simulink model "CombinedExperiment"  (R2020a)
settings: Solver=FixedStepAuto  StartTime=0.0  StopTime=tsim  FixedStep=baseRate  RelTol=1e-3  EnableMultiTasking=on
values from neighbouring files (symbols this model uses):
  baseRate = 0.1    [Run_Initializer.m]
  drop_states_BLACK = [1.36947387695313,1.22175756835938,-0.0161599479615688]    [Run_Initializer.m]
  drop_states_BLUE = [ xLength/2+0.9; yLength/2+0.5; 0]    [Run_Initializer.m]
  drop_states_RED = [ xLength/2+1.1; yLength/2; pi]    [Run_Initializer.m]
  F_thrusters_BLACK = 0.25.*ones(8,1)    [Run_Initializer.m]
  F_thrusters_BLUE = 0.25.*ones(8,1)    [Run_Initializer.m]
  F_thrusters_RED = 0.25.*ones(8,1)    [Run_Initializer.m]
  home_states_BLACK = [ xLength/2; yLength/2; 0]    [Run_Initializer.m]
  home_states_BLUE = [ xLength/2-0.9; yLength/2+0.5; 0]    [Run_Initializer.m]
  home_states_RED = [ xLength/2+1.1; yLength/2; pi]    [Run_Initializer.m]
  init_states_BLACK = [ xLength/2; yLength/2; 0]    [Run_Initializer.m]
  init_states_BLUE = [ xLength/2+0.9; yLength/2+0.5; 0]    [Run_Initializer.m]
  init_states_RED = [ xLength/2+1.1; yLength/2; pi]    [Run_Initializer.m]
  Kd_tb = 0.4    [Run_Initializer.m]
  Kd_tblue = 0.4    [Run_Initializer.m]
  Kd_tr = 0.4    [Run_Initializer.m]
  Kd_xb = 5    [Run_Initializer.m]
  Kd_xblue = 5    [Run_Initializer.m]
  Kd_xr = 5    [Run_Initializer.m]
  Kd_yb = 5    [Run_Initializer.m]
  Kd_yblue = 5    [Run_Initializer.m]
  Kd_yr = 5    [Run_Initializer.m]
  Kp_tb = 0.1    [Run_Initializer.m]
  Kp_tblue = 0.1    [Run_Initializer.m]
  Kp_tr = 0.1    [Run_Initializer.m]
  Kp_xb = 2    [Run_Initializer.m]
  Kp_xblue = 2    [Run_Initializer.m]
  Kp_xr = 2    [Run_Initializer.m]
  Kp_yb = 2    [Run_Initializer.m]
  Kp_yblue = 2    [Run_Initializer.m]
  Kp_yr = 2    [Run_Initializer.m]
  noise_variance_BLACK = 0    [Run_Initializer.m]
  noise_variance_BLUE = 0    [Run_Initializer.m]
  noise_variance_RED = 0    [Run_Initializer.m]
  Phase0_End = Phase0_Duration    (= 10)    [Run_Initializer.m]
  Phase1_End = Phase0_Duration + Phase1_Duration    (= 15)    [Run_Initializer.m]
  Phase2_End = Phase0_Duration + Phase1_Duration +                                   Phase2_Duration    (= 40)    [Run_Initializer.m]
  Phase3_End = Phase0_Duration + Phase1_Duration +                                   Phase2_Duration + Phase3_Duration    (= 117)    [Run_Initializer.m]
  Phase3_SubPhase1_End = Phase2_End + Phase3_SubPhase1_Duration    (= 41)    [Run_Initializer.m]
  Phase3_SubPhase2_End = Phase2_End + Phase3_SubPhase1_Duration +                                   Phase3_SubPhase2_Duration    (= 42)    [Run_Initializer.m]
  Phase3_SubPhase3_End = Phase2_End + Phase3_SubPhase1_Duration +                                   Phase3_SubPhase2_Duration +                                  Phase3_SubPhase3_Duration    (= 72)    [Run_Initializer.m]
  Phase3_SubPhase4_End = Phase2_End + Phase3_SubPhase1_Duration +                                   Phase3_SubPhase2_Duration +                                  Phase3_SubPhase3_Duration +                                  Phase3_SubPhase4_Duration    [Run_Initializer.m]
  Phase4_End = Phase0_Duration + Phase1_Duration +                                   Phase2_Duration + Phase3_Duration +                                   Phase4_Duration    (= 137)    [Run_Initializer.m]
  Phase5_End = Phase0_Duration + Phase1_Duration +                                   Phase2_Duration + Phase3_Duration +                                   Phase4_Duration + Phase5_Duration    (= 142)    [Run_Initializer.m]
  serverRate = 0.2    [Run_Initializer.m]
  thruster_dist2CG_BLACK = [83.42;-52.58;55.94;-60.05;54.08;-53.92;77.06;-55.94]    [Run_Initializer.m]
  thruster_dist2CG_BLUE = [83.42;-52.58;55.94;-60.05;54.08;-53.92;77.06;-55.94]    [Run_Initializer.m]
  thruster_dist2CG_RED = [49.92;-78.08;70.46;-63.54;81.08;-50.42;57.44;-75.96]    [Run_Initializer.m]
  xLength = 3.51155    [Run_Initializer.m]
  yLength = 2.41935    [Run_Initializer.m]
undefined symbols (not defined in the file or in its folder): DiscIntNeverNeededParam, platformSelection, simMode, WhoAmI
libraries: dspstat3 x18, raspberrypiBasiclib x10, dspsigops x9, embdlinuxlib x8, simulink x8, MainLibrary x5, mspfiltlib x3, dsparch4 x3, dspswit3 x2, sensehatlib x1
(part 4 of 9)

== system CombinedExperiment/From Force//Torque to PWM Signal/Change BLUE Behavior/Calculate Thruster ON//OFF ==
  note: Calculate which thrusters must be turned on and for how long.
  note: The H matrix is not square, thus a pserudo-inverse is required.
  note: Knowing how much force each thruster can output, we can determine the saturated thruster output and then convert is into a percentage of time over which each thruster is open.
  note: After finding the PWM value, we can use the H matrix to go back to torque and force. However, these torques and forces will be "saturated".
  "[Fx_b; Fy_b; Tz]" : Inport
  BLUE_Fx_Sat : DataStoreWrite  DataStoreName=BLUE_Fx_Sat
  BLUE_Fy_Sat : DataStoreWrite  DataStoreName=BLUE_Fy_Sat
  BLUE_Rz : DataStoreRead  DataStoreName=BLUE_Rz
  BLUE_Tz_Sat : DataStoreWrite  DataStoreName=BLUE_Tz_Sat
  Demux : Demux  Outputs=3
  Demux1 : Demux  Outputs=2
  MATLAB Function : MATLAB Function  TreatAsAtomicUnit=on
  MATLAB Function1 : MATLAB Function  TreatAsAtomicUnit=on
  MATLAB Function2 : MATLAB Function  TreatAsAtomicUnit=on
  Mux : Mux  Inputs=2
  Product : Product  Multiplication=Matrix(*)
  Product1 : Product  Multiplication=Matrix(*)
  Remove Negatives : Saturate  UpperLimit=1000  LowerLimit=0
  Rotate Forces to Inertial : Subsystem
  pseudo-inverse : Subsystem
  ThrusterPWM : Outport  VectorParamsAs1DForOutWhenUnconnected=off
  wires:
  pseudo-inverse/1(invH) -> Product/1
  Product/1 -> Remove Negatives/1
  "[Fx_b; Fy_b; Tz]"/1 -> Product/2
  MATLAB Function/1(H) -> pseudo-inverse/1(H)
  Remove Negatives/1 -> MATLAB Function2/1(ThrustPer)
  MATLAB Function1/1(H) -> Product1/1
  Product1/1 -> Demux/1
  Demux/2 -> Mux/2
  Demux/1 -> Mux/1
  Mux/1 -> Rotate Forces to Inertial/1("F_b ")
  BLUE_Rz/1 -> Rotate Forces to Inertial/2(Rz)
  Demux/3 -> BLUE_Tz_Sat/1
  Rotate Forces to Inertial/1(F_I) -> Demux1/1
  Demux1/1 -> BLUE_Fx_Sat/1
  Demux1/2 -> BLUE_Fy_Sat/1
  MATLAB Function2/1(ThrustPer_Final) -> Product1/2, ThrusterPWM/1

== system CombinedExperiment/From Force//Torque to PWM Signal/Change BLUE Behavior/Rotate Forces to Body ==
  "F_I " : Inport
  Rz : Inport  Port=2
  Create Rotation Matrix : MATLAB Function  TreatAsAtomicUnit=on
  Rotate F_I to F_b : Product  Multiplication=Matrix(*)
  F_b : Outport  VectorParamsAs1DForOutWhenUnconnected=off
  wires:
  Rotate F_I to F_b/1 -> F_b/1
  Create Rotation Matrix/1(C_bI) -> Rotate F_I to F_b/1
  "F_I "/1 -> Rotate F_I to F_b/2
  Rz/1 -> Create Rotation Matrix/1(Rz)

== system CombinedExperiment/From Force//Torque to PWM Signal/Change RED Behavior/Calculate Thruster ON//OFF ==
  note: Calculate which thrusters must be turned on and for how long.
  note: The H matrix is not square, thus a pserudo-inverse is required.
  note: Knowing how much force each thruster can output, we can determine the saturated thruster output and then convert is into a percentage of time over which each thruster is open.
  note: After finding the PWM value, we can use the H matrix to go back to torque and force. However, these torques and forces will be "saturated".
  "[Fx_b; Fy_b; Tz]" : Inport
  Demux : Demux  Outputs=3
  Demux1 : Demux  Outputs=2
  MATLAB Function : MATLAB Function  TreatAsAtomicUnit=on
  MATLAB Function1 : MATLAB Function  TreatAsAtomicUnit=on
  MATLAB Function2 : MATLAB Function  TreatAsAtomicUnit=on
  Mux : Mux  Inputs=2
  Product : Product  Multiplication=Matrix(*)
  Product1 : Product  Multiplication=Matrix(*)
  RED_Fx_Sat : DataStoreWrite  DataStoreName=RED_Fx_Sat
  RED_Fy_Sat : DataStoreWrite  DataStoreName=RED_Fy_Sat
  RED_Rz : DataStoreRead  DataStoreName=RED_Rz
  RED_Tz_Sat : DataStoreWrite  DataStoreName=RED_Tz_Sat
  Remove Negatives : Saturate  UpperLimit=1000  LowerLimit=0
  Rotate Forces to Inertial : Subsystem
  pseudo-inverse : Subsystem
  ThrusterPWM : Outport  VectorParamsAs1DForOutWhenUnconnected=off
  wires:
  pseudo-inverse/1(invH) -> Product/1
  Product/1 -> Remove Negatives/1
  "[Fx_b; Fy_b; Tz]"/1 -> Product/2
  MATLAB Function/1(H) -> pseudo-inverse/1(H)
  Remove Negatives/1 -> MATLAB Function2/1(ThrustPer)
  MATLAB Function1/1(H) -> Product1/1
  Product1/1 -> Demux/1
  Demux/2 -> Mux/2
  Demux/1 -> Mux/1
  Mux/1 -> Rotate Forces to Inertial/1("F_b ")
  RED_Rz/1 -> Rotate Forces to Inertial/2(Rz)
  Demux/3 -> RED_Tz_Sat/1
  Rotate Forces to Inertial/1(F_I) -> Demux1/1
  Demux1/1 -> RED_Fx_Sat/1
  Demux1/2 -> RED_Fy_Sat/1
  MATLAB Function2/1(ThrustPer_Final) -> Product1/2, ThrusterPWM/1

== system CombinedExperiment/From Force//Torque to PWM Signal/Change RED Behavior/Rotate Forces to Body ==
  "F_I " : Inport
  Rz : Inport  Port=2
  Create Rotation Matrix : MATLAB Function  TreatAsAtomicUnit=on
  Rotate F_I to F_b : Product  Multiplication=Matrix(*)
  F_b : Outport  VectorParamsAs1DForOutWhenUnconnected=off
  wires:
  Rotate F_I to F_b/1 -> F_b/1
  Create Rotation Matrix/1(C_bI) -> Rotate F_I to F_b/1
  "F_I "/1 -> Rotate F_I to F_b/2
  Rz/1 -> Create Rotation Matrix/1(Rz)

== system CombinedExperiment/From Torque, Command RW/Change RED Behavior/Calculate Saturated RPM Signal ==
  Tz : Inport
  Calculate RW RPM Increment : MATLAB Function  TreatAsAtomicUnit=on
  Delay : Delay  DelayLength=1
  Saturate RPM : Saturate  UpperLimit=(7000*64/3375)  LowerLimit=-(7000*64/3375)
  Saturate Torque : Saturate  UpperLimit=0.1  LowerLimit=-0.1
  Sum : Sum  Inputs=|++
  RPM : Outport  VectorParamsAs1DForOutWhenUnconnected=off
  RPM_Sat : Outport  Port=2  VectorParamsAs1DForOutWhenUnconnected=off
  wires:
  Tz/1 -> Saturate Torque/1
  Saturate RPM/1 -> Delay/1
  Calculate RW RPM Increment/1(dRPM_RW) -> Sum/1
  Delay/1 -> Sum/2
  Sum/1 -> RPM/1, Saturate RPM/1
  Saturate Torque/1 -> RPM_Sat/1, Calculate RW RPM Increment/1(Tz_Sat)

== system CombinedExperiment/From Torque, Command RW/Change RED Behavior/Wheel RPM to PWM ==
  note: Check the GPIO pin to see if the RW is ready to receive a command.
  note: Convert the RPM to a PWM value.
  note: Indicate Motor direction (0 for CW and 1 for CCW)
  WheelRPM : Inport
  Abs : Abs
  Check if RW is Ready : MATLAB Function  TreatAsAtomicUnit=on
  Convert Wheel Rate to Motor Rate : Subsystem
  Delay Bank : Subsystem
  Get RW Direction : MATLAB Function  TreatAsAtomicUnit=on
  Obtain RW Status : Subsystem  TreatAsAtomicUnit=on
  RED_RW_Speed : DataStoreWrite  DataStoreName=RED_dRz_RW_Sat
  RPM to PWM Value : MATLAB Function  TreatAsAtomicUnit=on
  Saturate Motor : Saturate  UpperLimit=7000  LowerLimit=-7000
  Send Direction to Motor Controller : Subsystem  TreatAsAtomicUnit=on
  Send PWM to Motor Controller : Subsystem  TreatAsAtomicUnit=on
  Turn on Motor : Subsystem  TreatAsAtomicUnit=on
  wires:
  WheelRPM/1 -> Check if RW is Ready/2(WheelRPM_In)
  Convert Wheel Rate to Motor Rate/1(Motor RPM) -> Saturate Motor/1
  Check if RW is Ready/2(WheelRPM_Out) -> RED_RW_Speed/1, Convert Wheel Rate to Motor Rate/1(Wheel RPM)
  Saturate Motor/1 -> Abs/1, Get RW Direction/1(MotorRPM_Sat)
  Delay Bank/1(StatusVector) -> Check if RW is Ready/1(Status)
  Abs/1 -> RPM to PWM Value/1(MotorRPM_Sat)
  Get RW Direction/1(WheelDirection) -> Send Direction to Motor Controller/1(WheelDir)
  RPM to PWM Value/1(MotorPWM) -> Send PWM to Motor Controller/1(MotorPWM)
  Obtain RW Status/1(RW_Status) -> Delay Bank/1(Status)
  Check if RW is Ready/1(EnableSig) -> Turn on Motor/1(EnableSig)

== system CombinedExperiment/Grab PhaseSpace Data via UDP/Use Hardware to Obtain States/Using RED+BLACK, or RED+BLACK+ARM ==
  note: In this subsection, the "if" statements are used to determine two things: 1) whether or not a simulation is begin performed,
      | then 2) if an experiment is being performed, then which platform is the diagram compiled on. The "IdentifyPlatform" variable
      | is obtained from a text file location on each platform; each text file contains a unique identifier for each platform.
  Action Port : ActionPort  ActionPortLabel=elseif(u1 == 3| u1 == 4)
  Constant : Constant  Value=WhoAmI
  Is this a simulation? : Subsystem
  Obtain BLACK States : Subsystem  TreatAsAtomicUnit=on
  Obtain RED States : Subsystem  TreatAsAtomicUnit=on
  This IF block determines whether or not to run the BLACK sim/exp : If  NumInputs=2  IfExpression=u1 == 2 | u2 == 1  ShowElse=off
  "This IF block determines whether or not to run the RED sim/exp " : If  NumInputs=2  IfExpression=u1 == 1 | u2 == 1  ShowElse=off
  wires:
  "This IF block determines whether or not to run the RED sim/exp "/1 -> Obtain RED States/Action
  Constant/1 -> This IF block determines whether or not to run the BLACK sim/exp/1, "This IF block determines whether or not to run the RED sim/exp "/1
  Is this a simulation?/1(isSim) -> This IF block determines whether or not to run the BLACK sim/exp/2, "This IF block determines whether or not to run the RED sim/exp "/2
  This IF block determines whether or not to run the BLACK sim/exp/1 -> Obtain BLACK States/Action

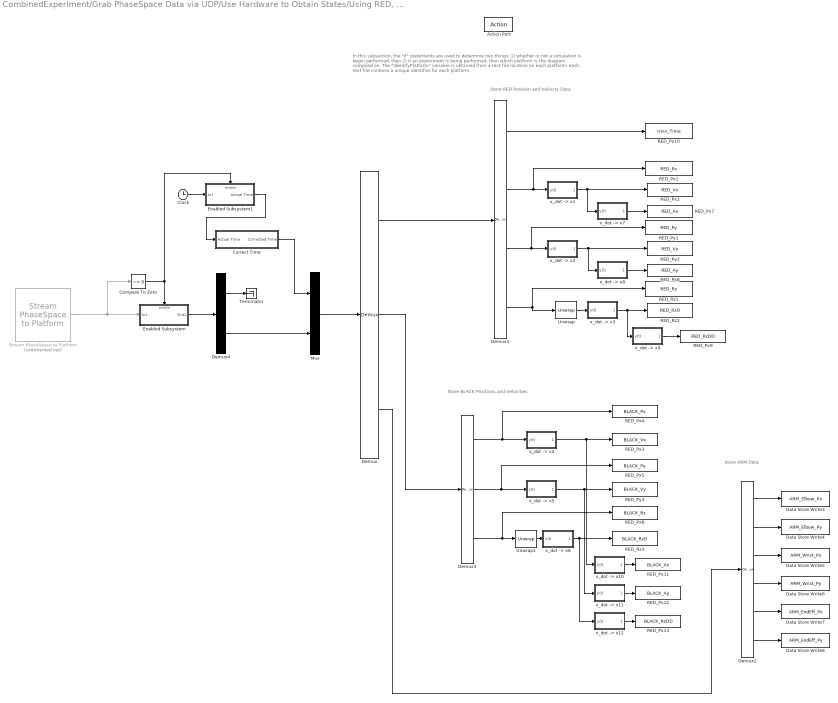
== system CombinedExperiment/Grab PhaseSpace Data via UDP/Use Hardware to Obtain States/Using RED, BLACK, BLUE, or RED + ARM ==
  note: In this subsection, the "if" statements are used to determine two things: 1) whether or not a simulation is begin performed,
      | then 2) if an experiment is being performed, then which platform is the diagram compiled on. The "IdentifyPlatform" variable
      | is obtained from a text file location on each platform; each text file contains a unique identifier for each platform.
  note: Store BLACK Positions and Velocities
  note: Store ARM Data
  note: Store RED Position and Velocity Data
  Action Port : ActionPort  ActionPortLabel=if(u1 == 1 | u1 == 2 | u1 == 5)
  Clock : Clock
  Compare To Zero : simulink/Logic and Bit Operations/Compare To Zero  relop=~=  OutDataTypeStr=boolean
  Correct Time : Subsystem
  Data Store Write3 : DataStoreWrite  DataStoreName=ARM_Elbow_Px
  Data Store Write4 : DataStoreWrite  DataStoreName=ARM_Elbow_Py
  Data Store Write5 : DataStoreWrite  DataStoreName=ARM_Wrist_Px
  Data Store Write6 : DataStoreWrite  DataStoreName=ARM_Wrist_Py
  Data Store Write7 : DataStoreWrite  DataStoreName=ARM_EndEff_Px
  Data Store Write8 : DataStoreWrite  DataStoreName=ARM_EndEff_Py
  Demux : Demux  Outputs=[4,3,6]
  Demux1 : Demux
  Demux2 : Demux  Outputs=6
  Demux3 : Demux  Outputs=3
  Demux4 : Demux  Outputs=[1,12]
  Enabled Subsystem : Subsystem  TreatAsAtomicUnit=on
  Enabled Subsystem1 : Subsystem  TreatAsAtomicUnit=on
  Mux : Mux  Inputs=2
  RED_Px1 : DataStoreWrite  DataStoreName=RED_Px
  RED_Px10 : DataStoreWrite  DataStoreName=Univ_Time
  RED_Px11 : DataStoreWrite  DataStoreName=BLACK_Ax
  RED_Px12 : DataStoreWrite  DataStoreName=BLACK_Ay
  RED_Px13 : DataStoreWrite  DataStoreName=BLACK_RzDD
  RED_Px2 : DataStoreWrite  DataStoreName=RED_Vx
  RED_Px3 : DataStoreWrite  DataStoreName=BLACK_Vx
  RED_Px4 : DataStoreWrite  DataStoreName=BLACK_Px
  RED_Px5 : DataStoreWrite  DataStoreName=BLACK_Py
  RED_Px6 : DataStoreWrite  DataStoreName=BLACK_Rz
  RED_Px7 : DataStoreWrite  DataStoreName=RED_Ax
  RED_Px8 : DataStoreWrite  DataStoreName=RED_Ay
  RED_Px9 : DataStoreWrite  DataStoreName=RED_RzDD
  RED_Py1 : DataStoreWrite  DataStoreName=RED_Py
  RED_Py2 : DataStoreWrite  DataStoreName=RED_Vy
  RED_Py3 : DataStoreWrite  DataStoreName=BLACK_Vy
  RED_Rz1 : DataStoreWrite  DataStoreName=RED_Rz
  RED_Rz2 : DataStoreWrite  DataStoreName=RED_RzD
  RED_Rz3 : DataStoreWrite  DataStoreName=BLACK_RzD
  Stream PhaseSpace to Platform : MainLibrary/PhaseSpace Functions/Stream PhaseSpace to Platform  Commented=on  platformSelection=platformSelection  PS_SampleRate=1/serverRate
      settings: SourceProductName=SPOT Custom Library
  Terminator : Terminator
  Unwrap : dspsigops/Unwrap  tol=pi  InputProcessing=Columns as channels (frame based)  running=off
  Unwrap1 : dspsigops/Unwrap  tol=pi  InputProcessing=Columns as channels (frame based)  running=off
  "x_dot -> x1" : Subsystem
  "x_dot -> x10" : Subsystem
  "x_dot -> x11" : Subsystem
  "x_dot -> x12" : Subsystem
  "x_dot -> x2" : Subsystem
  "x_dot -> x3" : Subsystem
  "x_dot -> x4" : Subsystem
  "x_dot -> x5" : Subsystem
  "x_dot -> x6" : Subsystem
  "x_dot -> x7" : Subsystem
  "x_dot -> x8" : Subsystem
  "x_dot -> x9" : Subsystem
  wires:
  "x_dot -> x8"/1(dy(t)/dt) -> RED_Px8/1
  Demux2/2 -> Data Store Write4/1
  Demux1/4 -> Unwrap/1, RED_Rz1/1
  Demux1/1 -> RED_Px10/1
  Unwrap/1 -> "x_dot -> x3"/1(y(t))
  "x_dot -> x7"/1(dy(t)/dt) -> RED_Px7/1
  Demux3/1 -> "x_dot -> x4"/1(y(t)), RED_Px4/1
  Unwrap1/1 -> "x_dot -> x6"/1(y(t))
  Demux/2 -> Demux3/1
  "x_dot -> x9"/1(dy(t)/dt) -> RED_Px9/1
  Demux/1 -> Demux1/1
  Demux/3 -> Demux2/1
  "x_dot -> x6"/1(dy(t)/dt) -> RED_Rz3/1, "x_dot -> x12"/1(y(t))
  "x_dot -> x3"/1(dy(t)/dt) -> "x_dot -> x9"/1(y(t)), RED_Rz2/1
  "x_dot -> x1"/1(dy(t)/dt) -> "x_dot -> x7"/1(y(t)), RED_Px2/1
  Demux1/2 -> "x_dot -> x1"/1(y(t)), RED_Px1/1
  Demux2/4 -> Data Store Write6/1
  Demux2/6 -> Data Store Write8/1
  "x_dot -> x2"/1(dy(t)/dt) -> "x_dot -> x8"/1(y(t)), RED_Py2/1
  Demux2/3 -> Data Store Write5/1
  Demux1/3 -> "x_dot -> x2"/1(y(t)), RED_Py1/1
  "x_dot -> x4"/1(dy(t)/dt) -> "x_dot -> x10"/1(y(t)), RED_Px3/1
  Demux2/1 -> Data Store Write3/1
  "x_dot -> x5"/1(dy(t)/dt) -> RED_Py3/1, "x_dot -> x11"/1(y(t))
  Demux2/5 -> Data Store Write7/1
  Demux3/3 -> Unwrap1/1, RED_Px6/1
  Demux3/2 -> "x_dot -> x5"/1(y(t)), RED_Px5/1
  "x_dot -> x10"/1(dy(t)/dt) -> RED_Px11/1
  "x_dot -> x11"/1(dy(t)/dt) -> RED_Px12/1
  "x_dot -> x12"/1(dy(t)/dt) -> RED_Px13/1
  Stream PhaseSpace to Platform/1 -> Enabled Subsystem/1(In1), Compare To Zero/1
  Enabled Subsystem/1(Out1) -> Demux4/1
  Compare To Zero/1 -> Enabled Subsystem1/Enable, Enabled Subsystem/Enable
  Demux4/2 -> Mux/2
  Mux/1 -> Demux/1
  Clock/1 -> Enabled Subsystem1/1(In1)
  Enabled Subsystem1/1(Actual Time) -> Correct Time/1(Actual Time)
  Correct Time/1(Corrected Time) -> Mux/1
  Demux4/1 -> Terminator/1

== system CombinedExperiment/Gyroscope & Acceleration Algorithms/Change BLACK Behavior/Fix Initial Bias ==
  Actual Gyro : Inport
  Correct GyroX : Subsystem
  Correct GyroY : Subsystem
  Correct GyroZ : Subsystem
  Demux : Demux  Outputs=3
  Mux : Mux  Inputs=3
  Corrected Gyro : Outport  VectorParamsAs1DForOutWhenUnconnected=off
  wires:
  Demux/1 -> Correct GyroX/1(In1)
  Demux/2 -> Correct GyroY/1(In1)
  Demux/3 -> Correct GyroZ/1(In1)
  Correct GyroX/1(Out1) -> Mux/1
  Correct GyroY/1(Out1) -> Mux/2
  Correct GyroZ/1(Out1) -> Mux/3
  Mux/1 -> Corrected Gyro/1
  Actual Gyro/1 -> Demux/1

== system CombinedExperiment/Gyroscope & Acceleration Algorithms/Change BLACK Behavior/Fix Initial Bias (Accel) ==
  Actual Accel : Inport
  Correct AccelX : Subsystem
  Correct AccelY : Subsystem
  Correct AccelZ : Subsystem
  Demux : Demux  Outputs=3
  Mux : Mux  Inputs=3
  Corrected Accel : Outport  VectorParamsAs1DForOutWhenUnconnected=off
  wires:
  Demux/1 -> Correct AccelX/1(In1)
  Demux/2 -> Correct AccelY/1(In1)
  Demux/3 -> Correct AccelZ/1(In1)
  Correct AccelX/1(Out1) -> Mux/1
  Correct AccelY/1(Out1) -> Mux/2
  Correct AccelZ/1(Out1) -> Mux/3
  Mux/1 -> Corrected Accel/1
  Actual Accel/1 -> Demux/1

== system CombinedExperiment/Gyroscope & Acceleration Algorithms/Change BLUE Behavior/Fix Initial Bias ==
  Actual Gyro : Inport
  Correct GyroX : Subsystem
  Correct GyroY : Subsystem
  Correct GyroZ : Subsystem
  Demux : Demux  Outputs=3
  Mux : Mux  Inputs=3
  Corrected Gyro : Outport  VectorParamsAs1DForOutWhenUnconnected=off
  wires:
  Demux/1 -> Correct GyroX/1(In1)
  Demux/2 -> Correct GyroY/1(In1)
  Demux/3 -> Correct GyroZ/1(In1)
  Correct GyroX/1(Out1) -> Mux/1
  Correct GyroY/1(Out1) -> Mux/2
  Correct GyroZ/1(Out1) -> Mux/3
  Mux/1 -> Corrected Gyro/1
  Actual Gyro/1 -> Demux/1

== system CombinedExperiment/Gyroscope & Acceleration Algorithms/Change BLUE Behavior/Fix Initial Bias (Accel) ==
  Actual Accel : Inport
  Correct AccelX : Subsystem
  Correct AccelY : Subsystem
  Correct AccelZ : Subsystem
  Demux : Demux  Outputs=3
  Mux : Mux  Inputs=3
  Corrected Accel : Outport  VectorParamsAs1DForOutWhenUnconnected=off
  wires:
  Demux/1 -> Correct AccelX/1(In1)
  Demux/2 -> Correct AccelY/1(In1)
  Demux/3 -> Correct AccelZ/1(In1)
  Correct AccelX/1(Out1) -> Mux/1
  Correct AccelY/1(Out1) -> Mux/2
  Correct AccelZ/1(Out1) -> Mux/3
  Mux/1 -> Corrected Accel/1
  Actual Accel/1 -> Demux/1

== system CombinedExperiment/Gyroscope & Acceleration Algorithms/Change RED Behavior/Fix Initial Bias ==
  Actual Gyro : Inport
  Correct GyroX : Subsystem
  Correct GyroY : Subsystem
  Correct GyroZ : Subsystem
  Demux : Demux  Outputs=3
  Mux : Mux  Inputs=3
  Corrected Gyro : Outport  VectorParamsAs1DForOutWhenUnconnected=off
  wires:
  Demux/1 -> Correct GyroX/1(In1)
  Demux/2 -> Correct GyroY/1(In1)
  Demux/3 -> Correct GyroZ/1(In1)
  Correct GyroX/1(Out1) -> Mux/1
  Correct GyroY/1(Out1) -> Mux/2
  Correct GyroZ/1(Out1) -> Mux/3
  Mux/1 -> Corrected Gyro/1
  Actual Gyro/1 -> Demux/1

== system CombinedExperiment/Gyroscope & Acceleration Algorithms/Change RED Behavior/Fix Initial Bias (Accel) ==
  Actual Accel : Inport
  Correct AccelX : Subsystem
  Correct AccelY : Subsystem
  Correct AccelZ : Subsystem
  Demux : Demux  Outputs=3
  Mux : Mux  Inputs=3
  Corrected Accel : Outport  VectorParamsAs1DForOutWhenUnconnected=off
  wires:
  Demux/1 -> Correct AccelX/1(In1)
  Demux/2 -> Correct AccelY/1(In1)
  Demux/3 -> Correct AccelZ/1(In1)
  Correct AccelX/1(Out1) -> Mux/1
  Correct AccelY/1(Out1) -> Mux/2
  Correct AccelZ/1(Out1) -> Mux/3
  Mux/1 -> Corrected Accel/1
  Actual Accel/1 -> Demux/1

== system CombinedExperiment/Phase #2: Move to Initial Position/Change BLACK Behavior/Custom Discrete PD (Attitude) ==
  ez : Inport
  Sum3 : Sum
  kd_tb : Gain  Gain=Kd_tb
  kp_tb : Gain  Gain=Kp_tb
  "x_dot -> x1" : Subsystem
  Tz : Outport  VectorParamsAs1DForOutWhenUnconnected=off
  wires:
  kd_tb/1 -> Sum3/1
  Sum3/1 -> Tz/1
  kp_tb/1 -> Sum3/2
  "x_dot -> x1"/1(dy(t)/dt) -> kd_tb/1
  ez/1 -> "x_dot -> x1"/1(y(t)), kp_tb/1

== system CombinedExperiment/Phase #2: Move to Initial Position/Change BLACK Behavior/Custom Discrete PD (X-Position) ==
  ex : Inport
  Sum3 : Sum
  kd_xb : Gain  Gain=Kd_xb
  kp_xb : Gain  Gain=Kp_xb
  "x_dot -> x1" : Subsystem
  Fx : Outport  VectorParamsAs1DForOutWhenUnconnected=off
  wires:
  kd_xb/1 -> Sum3/1
  ex/1 -> "x_dot -> x1"/1(y(t)), kp_xb/1
  kp_xb/1 -> Sum3/2
  "x_dot -> x1"/1(dy(t)/dt) -> kd_xb/1
  Sum3/1 -> Fx/1

== system CombinedExperiment/Phase #2: Move to Initial Position/Change BLACK Behavior/Custom Discrete PD (Y-Position) ==
  ey : Inport
  Sum3 : Sum
  kd_yb : Gain  Gain=Kd_yb
  kp_yb : Gain  Gain=Kp_yb
  "x_dot -> x1" : Subsystem
  Fy : Outport  VectorParamsAs1DForOutWhenUnconnected=off
  wires:
  kd_yb/1 -> Sum3/1
  Sum3/1 -> Fy/1
  kp_yb/1 -> Sum3/2
  "x_dot -> x1"/1(dy(t)/dt) -> kd_yb/1
  ey/1 -> "x_dot -> x1"/1(y(t)), kp_yb/1

== system CombinedExperiment/Phase #2: Move to Initial Position/Change BLACK Behavior/Hough Control ==
  Ref : Inport
  Act : Inport  Port=2
  MATLAB Function2 : MATLAB Function  TreatAsAtomicUnit=on
  MATLAB Function3 : MATLAB Function  TreatAsAtomicUnit=on
  MATLAB Function4 : MATLAB Function  TreatAsAtomicUnit=on
  Subtract2 : Sum  Inputs=+-
  Err : Outport  VectorParamsAs1DForOutWhenUnconnected=off
  wires:
  MATLAB Function4/1(e_out) -> Err/1
  MATLAB Function2/1(Oy) -> MATLAB Function4/1(Oy)
  Subtract2/1 -> MATLAB Function4/2(e_in)
  MATLAB Function2/2(Ox) -> Subtract2/1
  Act/1 -> MATLAB Function3/1(z)
  Ref/1 -> MATLAB Function2/1(z)
  MATLAB Function3/1(Ox) -> Subtract2/2

== system CombinedExperiment/Phase #2: Move to Initial Position/Change BLUE Behavior/Custom Discrete PD (Attitude) ==
  ez : Inport
  Sum3 : Sum
  kd_tb : Gain  Gain=Kd_tblue
  kp_tb : Gain  Gain=Kp_tblue
  "x_dot -> x1" : Subsystem
  Tz : Outport  VectorParamsAs1DForOutWhenUnconnected=off
  wires:
  kd_tb/1 -> Sum3/1
  Sum3/1 -> Tz/1
  kp_tb/1 -> Sum3/2
  "x_dot -> x1"/1(dy(t)/dt) -> kd_tb/1
  ez/1 -> "x_dot -> x1"/1(y(t)), kp_tb/1

== system CombinedExperiment/Phase #2: Move to Initial Position/Change BLUE Behavior/Custom Discrete PD (X-Position) ==
  ex : Inport
  Sum3 : Sum
  kd_xb : Gain  Gain=Kd_xblue
  kp_xb : Gain  Gain=Kp_xblue
  "x_dot -> x1" : Subsystem
  Fx : Outport  VectorParamsAs1DForOutWhenUnconnected=off
  wires:
  kd_xb/1 -> Sum3/1
  ex/1 -> "x_dot -> x1"/1(y(t)), kp_xb/1
  kp_xb/1 -> Sum3/2
  "x_dot -> x1"/1(dy(t)/dt) -> kd_xb/1
  Sum3/1 -> Fx/1

== system CombinedExperiment/Phase #2: Move to Initial Position/Change BLUE Behavior/Custom Discrete PD (Y-Position) ==
  ey : Inport
  Sum3 : Sum
  kd_yb : Gain  Gain=Kd_yblue
  kp_yb : Gain  Gain=Kp_yblue
  "x_dot -> x1" : Subsystem
  Fy : Outport  VectorParamsAs1DForOutWhenUnconnected=off
  wires:
  kd_yb/1 -> Sum3/1
  Sum3/1 -> Fy/1
  kp_yb/1 -> Sum3/2
  "x_dot -> x1"/1(dy(t)/dt) -> kd_yb/1
  ey/1 -> "x_dot -> x1"/1(y(t)), kp_yb/1

== system CombinedExperiment/Phase #2: Move to Initial Position/Change BLUE Behavior/Hough Control ==
  Ref : Inport
  Act : Inport  Port=2
  MATLAB Function2 : MATLAB Function  TreatAsAtomicUnit=on
  MATLAB Function3 : MATLAB Function  TreatAsAtomicUnit=on
  MATLAB Function4 : MATLAB Function  TreatAsAtomicUnit=on
  Subtract2 : Sum  Inputs=+-
  Err : Outport  VectorParamsAs1DForOutWhenUnconnected=off
  wires:
  MATLAB Function4/1(e_out) -> Err/1
  MATLAB Function2/1(Oy) -> MATLAB Function4/1(Oy)
  Subtract2/1 -> MATLAB Function4/2(e_in)
  MATLAB Function2/2(Ox) -> Subtract2/1
  Act/1 -> MATLAB Function3/1(z)
  Ref/1 -> MATLAB Function2/1(z)
  MATLAB Function3/1(Ox) -> Subtract2/2

== system CombinedExperiment/Phase #2: Move to Initial Position/Change RED Behavior/Custom Discrete PD (Attitude) ==
  ez : Inport
  Sum3 : Sum
  kd_tr : Gain  Gain=Kd_tr
  kp_tr : Gain  Gain=Kp_tr
  "x_dot -> x1" : Subsystem
  Tz : Outport  VectorParamsAs1DForOutWhenUnconnected=off
  wires:
  kd_tr/1 -> Sum3/1
  Sum3/1 -> Tz/1
  kp_tr/1 -> Sum3/2
  "x_dot -> x1"/1(dy(t)/dt) -> kd_tr/1
  ez/1 -> "x_dot -> x1"/1(y(t)), kp_tr/1

== system CombinedExperiment/Phase #2: Move to Initial Position/Change RED Behavior/Custom Discrete PD (X-Position) ==
  ex : Inport
  Sum3 : Sum
  kd_xr : Gain  Gain=Kd_xr
  kp_xr : Gain  Gain=Kp_xr
  "x_dot -> x1" : Subsystem
  Fx : Outport  VectorParamsAs1DForOutWhenUnconnected=off
  wires:
  kd_xr/1 -> Sum3/1
  ex/1 -> "x_dot -> x1"/1(y(t)), kp_xr/1
  kp_xr/1 -> Sum3/2
  "x_dot -> x1"/1(dy(t)/dt) -> kd_xr/1
  Sum3/1 -> Fx/1

== system CombinedExperiment/Phase #2: Move to Initial Position/Change RED Behavior/Custom Discrete PD (Y-Position) ==
  ey : Inport
  Sum3 : Sum
  kd_yr : Gain  Gain=Kd_yr
  kp_yr : Gain  Gain=Kp_yr
  "x_dot -> x1" : Subsystem
  Fy : Outport  VectorParamsAs1DForOutWhenUnconnected=off
  wires:
  kd_yr/1 -> Sum3/1
  Sum3/1 -> Fy/1
  kp_yr/1 -> Sum3/2
  "x_dot -> x1"/1(dy(t)/dt) -> kd_yr/1
  ey/1 -> "x_dot -> x1"/1(y(t)), kp_yr/1

== system CombinedExperiment/Phase #2: Move to Initial Position/Change RED Behavior/Hough Control ==
  Ref : Inport
  Act : Inport  Port=2
  MATLAB Function2 : MATLAB Function  TreatAsAtomicUnit=on
  MATLAB Function3 : MATLAB Function  TreatAsAtomicUnit=on
  MATLAB Function4 : MATLAB Function  TreatAsAtomicUnit=on
  Subtract2 : Sum  Inputs=+-
  Err : Outport  VectorParamsAs1DForOutWhenUnconnected=off
  wires:
  MATLAB Function4/1(e_out) -> Err/1
  MATLAB Function2/1(Oy) -> MATLAB Function4/1(Oy)
  Subtract2/1 -> MATLAB Function4/2(e_in)
  MATLAB Function2/2(Ox) -> Subtract2/1
  Act/1 -> MATLAB Function3/1(z)
  Ref/1 -> MATLAB Function2/1(z)
  MATLAB Function3/1(Ox) -> Subtract2/2

== system CombinedExperiment/Phase #3: Experiment/Change BLACK Behavior/Sub-Phase #1 ==
  note: PD Control Law - BLACK
  note: Additional Blocks
  note: A simple PD control law is used here to command the platform to it's initial position, as defined in the initializer.
  note: Additional blocks are stored here.
  Action Port : ActionPort  ActionPortLabel=if(u1 < u2)
  BLACK_Fx : DataStoreWrite  DataStoreName=BLACK_Fx
  BLACK_Fy : DataStoreWrite  DataStoreName=BLACK_Fy
  BLACK_Px : DataStoreRead  DataStoreName=BLACK_Px
  "BLACK_Py " : DataStoreRead  DataStoreName=BLACK_Py
  BLACK_Rz : DataStoreRead  DataStoreName=BLACK_Rz
  BLACK_Tz : DataStoreWrite  DataStoreName=BLACK_Tz
  Custom Discrete PD (Attitude) : Subsystem
  Custom Discrete PD (X-Position) : Subsystem
  Custom Discrete PD (Y-Position) : Subsystem
  Data Store Write3 : DataStoreWrite  DataStoreName=Float_State
  Desired Attitude (BLACK) : Constant  Value=init_states_BLACK(3)  SampleTime=-1
  Desired X-Position (BLACK) : Constant  Value=init_states_BLACK(1)  SampleTime=-1
  Desired Y-Position (BLACK) : Constant  Value=init_states_BLACK(2)  SampleTime=-1
  Hough Control : Subsystem
  Puck State : Constant
  Subtract : Sum  Inputs=+-
  Subtract1 : Sum  Inputs=+-
  wires:
  BLACK_Rz/1 -> Hough Control/2(Act)
  Subtract/1 -> Custom Discrete PD (X-Position)/1(ex)
  Desired Y-Position (BLACK)/1 -> Subtract1/1
  BLACK_Px/1 -> Subtract/2
  Custom Discrete PD (Y-Position)/1(Fy) -> BLACK_Fy/1
  Custom Discrete PD (Attitude)/1(Tz) -> BLACK_Tz/1
  Desired X-Position (BLACK)/1 -> Subtract/1
  "BLACK_Py "/1 -> Subtract1/2
  Subtract1/1 -> Custom Discrete PD (Y-Position)/1(ey)
  Hough Control/1(Err) -> Custom Discrete PD (Attitude)/1(ez)
  Desired Attitude (BLACK)/1 -> Hough Control/1(Ref)
  Custom Discrete PD (X-Position)/1(Fx) -> BLACK_Fx/1
  Puck State/1 -> Data Store Write3/1

== system CombinedExperiment/Phase #3: Experiment/Change BLACK Behavior/Sub-Phase #2  ==
  note: PD Control Law - BLACK
  note: Additional Blocks
  note: Additional blocks are stored here.
  Action Port : ActionPort  ActionPortLabel=elseif(u1 < u3)
  BLACK_Fx : DataStoreWrite  DataStoreName=BLACK_Fx
  BLACK_Fy : DataStoreWrite  DataStoreName=BLACK_Fy
  BLACK_Tz : DataStoreWrite  DataStoreName=BLACK_Tz
  Constant : Constant  Value=0
  Data Store Write3 : DataStoreWrite  DataStoreName=Float_State
  Puck State : Constant  Value=0
  wires:
  Constant/1 -> BLACK_Tz/1, BLACK_Fx/1, BLACK_Fy/1
  Puck State/1 -> Data Store Write3/1

== system CombinedExperiment/Phase #3: Experiment/Change BLACK Behavior/Sub-Phase #3  ==
  note: PD Control Law - BLACK
  note: Additional Blocks
  note: Additional blocks are stored here.
  Action Port : ActionPort  ActionPortLabel=elseif( u1 < u4)
  BLACK_Fx : DataStoreWrite  DataStoreName=BLACK_Fx
  BLACK_Fy : DataStoreWrite  DataStoreName=BLACK_Fy
  BLACK_Tz : DataStoreWrite  DataStoreName=BLACK_Tz
  Constant : Constant  Value=0
  Data Store Write3 : DataStoreWrite  DataStoreName=Float_State
  Puck State : Constant  Value=0
  wires:
  Constant/1 -> BLACK_Tz/1, BLACK_Fx/1, BLACK_Fy/1
  Puck State/1 -> Data Store Write3/1

== system CombinedExperiment/Phase #3: Experiment/Change BLACK Behavior/Sub-Phase #4 ==
  note: PD Control Law - BLACK
  note: Additional Blocks
  note: A simple PD control law is used here to command the platform to it's initial position, as defined in the initializer.
  note: Additional blocks are stored here.
  Action Port : ActionPort  ActionPortLabel=elseif( u1 < u5)
  BLACK_Fx : DataStoreWrite  DataStoreName=BLACK_Fx
  BLACK_Fy : DataStoreWrite  DataStoreName=BLACK_Fy
  BLACK_Px : DataStoreRead  DataStoreName=BLACK_Px
  "BLACK_Py " : DataStoreRead  DataStoreName=BLACK_Py
  BLACK_Rz : DataStoreRead  Commented=on  DataStoreName=BLACK_Rz
  BLACK_RzD : Subsystem  Commented=on
  BLACK_RzD1 : Subsystem  Commented=on
  BLACK_Tz : DataStoreWrite  Commented=on  DataStoreName=BLACK_Tz
  Custom Discrete PD (Attitude) : Subsystem  Commented=on
  Custom Discrete PD (X-Position) : Subsystem
  Custom Discrete PD (Y-Position) : Subsystem
  Data Store Write3 : DataStoreWrite  DataStoreName=Float_State
  Desired X-Position (BLACK) : Constant  Value=xLength/2  SampleTime=-1
  Desired Y-Position (BLACK) : Constant  Value=yLength/2  SampleTime=-1
  Hough Control : Subsystem  Commented=on
  Puck State : Constant
  Subtract : Sum  Inputs=+-
  Subtract1 : Sum  Inputs=+-
  wires:
  "BLACK_Py "/1 -> Subtract1/2
  Subtract1/1 -> Custom Discrete PD (Y-Position)/1(ey)
  Desired Y-Position (BLACK)/1 -> Subtract1/1
  Custom Discrete PD (Y-Position)/1(Fy) -> BLACK_Fy/1
  Desired X-Position (BLACK)/1 -> Subtract/1
  Custom Discrete PD (Attitude)/1(Tz) -> BLACK_Tz/1
  Hough Control/1(Err) -> Custom Discrete PD (Attitude)/1(ez)
  Puck State/1 -> Data Store Write3/1
  BLACK_Rz/1 -> Hough Control/2(Act)
  BLACK_Px/1 -> Subtract/2
  Custom Discrete PD (X-Position)/1(Fx) -> BLACK_Fx/1
  Subtract/1 -> Custom Discrete PD (X-Position)/1(ex)
  BLACK_RzD1/1(Out1) -> Hough Control/1(Ref)

== system CombinedExperiment/Phase #3: Experiment/Change BLACK Behavior/Subsystem ==
  Universal_Time : DataStoreRead  DataStoreName=Univ_Time
  Time : Outport  VectorParamsAs1DForOutWhenUnconnected=off
  wires:
  Universal_Time/1 -> Time/1

== system CombinedExperiment/Phase #3: Experiment/Change BLUE Behavior/Sub-Phase #1 ==
  note: PD Control Law - BLUE
  note: A simple PD control law is used here to command the platform to it's initial position, as defined in the initializer.
  note: Additional Blocks
  note: Additional blocks are stored here.
  Action Port : ActionPort  ActionPortLabel=if(u1 < u2)
  BLUE_Fx : DataStoreWrite  DataStoreName=BLUE_Fx
  BLUE_Fy : DataStoreWrite  DataStoreName=BLUE_Fy
  BLUE_Px : DataStoreRead  DataStoreName=BLUE_Px
  "BLUE_Py " : DataStoreRead  DataStoreName=BLUE_Py
  BLUE_Rz : DataStoreRead  DataStoreName=BLUE_Rz
  BLUE_Tz : DataStoreWrite  DataStoreName=BLUE_Tz
  Custom Discrete PD (Attitude) : Subsystem
  Custom Discrete PD (X-Position) : Subsystem
  Custom Discrete PD (Y-Position) : Subsystem
  Data Store Write1 : DataStoreWrite  DataStoreName=Float_State
  Desired Attitude (BLUE) : Constant  Value=init_states_BLUE(3)  SampleTime=-1
  Desired Px (BLUE) : Constant  Value=init_states_BLUE(1)  SampleTime=-1
  Desired Py (BLUE) : Constant  Value=init_states_BLUE(2)  SampleTime=-1
  Hough Control : Subsystem
  Puck State : Constant
  Subtract : Sum  Inputs=+-
  Subtract1 : Sum  Inputs=+-
  wires:
  Puck State/1 -> Data Store Write1/1
  Subtract/1 -> Custom Discrete PD (X-Position)/1(ex)
  Desired Py (BLUE)/1 -> Subtract1/1
  Custom Discrete PD (X-Position)/1(Fx) -> BLUE_Fx/1
  Desired Px (BLUE)/1 -> Subtract/1
  Subtract1/1 -> Custom Discrete PD (Y-Position)/1(ey)
  Hough Control/1(Err) -> Custom Discrete PD (Attitude)/1(ez)
  Desired Attitude (BLUE)/1 -> Hough Control/1(Ref)
  Custom Discrete PD (Attitude)/1(Tz) -> BLUE_Tz/1
  "BLUE_Py "/1 -> Subtract1/2
  Custom Discrete PD (Y-Position)/1(Fy) -> BLUE_Fy/1
  BLUE_Px/1 -> Subtract/2
  BLUE_Rz/1 -> Hough Control/2(Act)

== system CombinedExperiment/Phase #3: Experiment/Change BLUE Behavior/Sub-Phase #2  ==
  note: Additional blocks are stored here.
  note: A simple PD control law is used here to command the platform to it's initial position, as defined in the initializer.
  note: Additional Blocks
  note: PD Control Law - BLUE
  Action Port : ActionPort  ActionPortLabel=elseif(u1 < u3)
  BLUE_Fx : DataStoreWrite  DataStoreName=BLUE_Fx
  BLUE_Fy : DataStoreWrite  DataStoreName=BLUE_Fy
  BLUE_Tz : DataStoreWrite  DataStoreName=BLUE_Tz
  Constant : Constant  Value=0
  Data Store Write1 : DataStoreWrite  DataStoreName=Float_State
  Puck State : Constant  Value=0
  wires:
  Puck State/1 -> Data Store Write1/1
  Constant/1 -> BLUE_Tz/1, BLUE_Fx/1, BLUE_Fy/1

== system CombinedExperiment/Phase #3: Experiment/Change BLUE Behavior/Sub-Phase #3  ==
  note: Additional blocks are stored here.
  note: A simple PD control law is used here to command the platform to it's initial position, as defined in the initializer.
  note: Additional Blocks
  note: PD Control Law - BLUE
  Action Port : ActionPort  ActionPortLabel=elseif( u1 < u4)
  BLUE_Fx : DataStoreWrite  DataStoreName=BLUE_Fx
  BLUE_Fy : DataStoreWrite  DataStoreName=BLUE_Fy
  BLUE_Tz : DataStoreWrite  DataStoreName=BLUE_Tz
  Constant : Constant  Value=0
  Data Store Write1 : DataStoreWrite  DataStoreName=Float_State
  Puck State : Constant
  wires:
  Constant/1 -> BLUE_Tz/1, BLUE_Fx/1, BLUE_Fy/1
  Puck State/1 -> Data Store Write1/1

== system CombinedExperiment/Phase #3: Experiment/Change BLUE Behavior/Sub-Phase #4 ==
  note: Additional blocks are stored here.
  note: A simple PD control law is used here to command the platform to it's initial position, as defined in the initializer.
  note: Additional Blocks
  note: PD Control Law - BLUE
  Action Port : ActionPort  ActionPortLabel=elseif( u1 < u5)
  BLUE_Fx : DataStoreWrite  DataStoreName=BLUE_Fx
  BLUE_Fy : DataStoreWrite  DataStoreName=BLUE_Fy
  BLUE_Px : DataStoreRead  DataStoreName=BLUE_Px
  "BLUE_Py " : DataStoreRead  DataStoreName=BLUE_Py
  BLUE_Rz : DataStoreRead  DataStoreName=BLUE_Rz
  BLUE_Tz : DataStoreWrite  DataStoreName=BLUE_Tz
  Custom Discrete PD (Attitude) : Subsystem
  Custom Discrete PD (X-Position) : Subsystem
  Custom Discrete PD (Y-Position) : Subsystem
  Data Store Write1 : DataStoreWrite  DataStoreName=Float_State
  Desired Attitude (BLUE) : Constant  Value=init_states_BLUE(3)  SampleTime=-1
  Desired Px (BLUE) : Constant  Value=init_states_BLUE(1)  SampleTime=-1
  Desired Py (BLUE) : Constant  Value=init_states_BLUE(2)  SampleTime=-1
  Hough Control : Subsystem
  Puck State : Constant
  Subtract : Sum  Inputs=+-
  Subtract1 : Sum  Inputs=+-
  wires:
  Puck State/1 -> Data Store Write1/1
  Subtract/1 -> Custom Discrete PD (X-Position)/1(ex)
  Desired Py (BLUE)/1 -> Subtract1/1
  Custom Discrete PD (X-Position)/1(Fx) -> BLUE_Fx/1
  Desired Px (BLUE)/1 -> Subtract/1
  Subtract1/1 -> Custom Discrete PD (Y-Position)/1(ey)
  Hough Control/1(Err) -> Custom Discrete PD (Attitude)/1(ez)
  Desired Attitude (BLUE)/1 -> Hough Control/1(Ref)
  Custom Discrete PD (Attitude)/1(Tz) -> BLUE_Tz/1
  "BLUE_Py "/1 -> Subtract1/2
  Custom Discrete PD (Y-Position)/1(Fy) -> BLUE_Fy/1
  BLUE_Px/1 -> Subtract/2
  BLUE_Rz/1 -> Hough Control/2(Act)

== system CombinedExperiment/Phase #3: Experiment/Change BLUE Behavior/Subsystem ==
  Universal_Time : DataStoreRead  DataStoreName=Univ_Time
  Time : Outport  VectorParamsAs1DForOutWhenUnconnected=off
  wires:
  Universal_Time/1 -> Time/1

== system CombinedExperiment/Phase #3: Experiment/Change RED Behavior/Sub-Phase #1 ==
  note: ARM Control Law - RED
  note: This section is reserved for any control law for the robotic manipulator.
  note: Additional Blocks
  note: PD Control Law - RED
  note: Additional blocks are stored above. Note that to control attitude using the RW, simply replace RED_Tz with RED_Tz_RW.
  Action Port : ActionPort  ActionPortLabel=if(u1 < u2)
  Constant{,1,4..6} (5 alike) : Constant  Value=0
  Data Store Write : DataStoreWrite  DataStoreName=RED_Tz_Shoulder
  Data Store Write1 : DataStoreWrite  DataStoreName=RED_Tz_Elbow
  Data Store Write2 : DataStoreWrite  DataStoreName=RED_Tz_Wrist
  Data Store Write3 : DataStoreWrite  DataStoreName=Float_State
  Puck State : Constant  Value=0
  RED_Fx : DataStoreWrite  DataStoreName=RED_Fx
  RED_Fy : DataStoreWrite  DataStoreName=RED_Fy
  RED_Tz : DataStoreWrite  DataStoreName=RED_Tz
  RED_Tz_RW : DataStoreWrite  DataStoreName=RED_Tz_RW
  wires:
  Constant/1 -> RED_Tz/1, RED_Fx/1, RED_Fy/1
  Constant6/1 -> Data Store Write2/1
  Puck State/1 -> Data Store Write3/1
  Constant4/1 -> Data Store Write/1
  Constant5/1 -> Data Store Write1/1
  Constant1/1 -> RED_Tz_RW/1

== system CombinedExperiment/Phase #3: Experiment/Change RED Behavior/Sub-Phase #2  ==
  note: ARM Control Law - RED
  note: PD Control Law - RED
  note: Additional Blocks
  note: Additional blocks are stored above. Note that to control attitude using the RW, simply replace RED_Tz with RED_Tz_RW.
  note: This section is reserved for any control law for the robotic manipulator.
  Action Port : ActionPort  ActionPortLabel=elseif(u1 < u3)
  Constant{,1,4..6} (5 alike) : Constant  Value=0
  Data Store Write : DataStoreWrite  DataStoreName=RED_Tz_Shoulder
  Data Store Write1 : DataStoreWrite  DataStoreName=RED_Tz_Elbow
  Data Store Write2 : DataStoreWrite  DataStoreName=RED_Tz_Wrist
  Data Store Write3 : DataStoreWrite  DataStoreName=Float_State
  Puck State : Constant
  RED_Fx : DataStoreWrite  DataStoreName=RED_Fx
  RED_Fy : DataStoreWrite  DataStoreName=RED_Fy
  RED_Tz : DataStoreWrite  DataStoreName=RED_Tz
  RED_Tz_RW : DataStoreWrite  DataStoreName=RED_Tz_RW
  wires:
  Constant1/1 -> RED_Tz_RW/1
  Constant6/1 -> Data Store Write2/1
  Constant4/1 -> Data Store Write/1
  Constant5/1 -> Data Store Write1/1
  Constant/1 -> RED_Tz/1, RED_Fx/1, RED_Fy/1
  Puck State/1 -> Data Store Write3/1

== system CombinedExperiment/Phase #3: Experiment/Change RED Behavior/Sub-Phase #3  ==
  note: ARM Control Law - RED
  note: PD Control Law - RED
  note: Additional Blocks
  note: Additional blocks are stored above. Note that to control attitude using the RW, simply replace RED_Tz with RED_Tz_RW.
  note: This section is reserved for any control law for the robotic manipulator.
  Action Port : ActionPort  ActionPortLabel=elseif( u1 < u4)
  Constant{,1,4..6} (5 alike) : Constant  Value=0
  Data Store Write : DataStoreWrite  DataStoreName=RED_Tz_Shoulder
  Data Store Write1 : DataStoreWrite  DataStoreName=RED_Tz_Elbow
  Data Store Write2 : DataStoreWrite  DataStoreName=RED_Tz_Wrist
  Data Store Write3 : DataStoreWrite  DataStoreName=Float_State
  From Workspace : FromWorkspace  VariableName=Pos_J1  SampleTime=-1
  From Workspace1 : FromWorkspace  VariableName=Pos_J2  SampleTime=-1
  From Workspace2 : FromWorkspace  VariableName=Pos_J3  SampleTime=-1
  Puck State : Constant
  RED_Fx : DataStoreWrite  DataStoreName=RED_Fx
  RED_Fy : DataStoreWrite  DataStoreName=RED_Fy
  RED_Tz : DataStoreWrite  DataStoreName=RED_Tz
  RED_Tz_RW : DataStoreWrite  DataStoreName=RED_Tz_RW
  Send Position Commands to Manipulator : MainLibrary/Dynamixel Functions/Send Position Commands to Manipulator
      settings: SourceProductName=SPOT Custom Library
  wires:
  Constant1/1 -> RED_Tz_RW/1
  Constant6/1 -> Data Store Write2/1
  Constant4/1 -> Data Store Write/1
  Constant5/1 -> Data Store Write1/1
  Constant/1 -> RED_Tz/1, RED_Fx/1, RED_Fy/1
  Puck State/1 -> Data Store Write3/1
  From Workspace2/1 -> Send Position Commands to Manipulator/3
  From Workspace1/1 -> Send Position Commands to Manipulator/2
  From Workspace/1 -> Send Position Commands to Manipulator/1

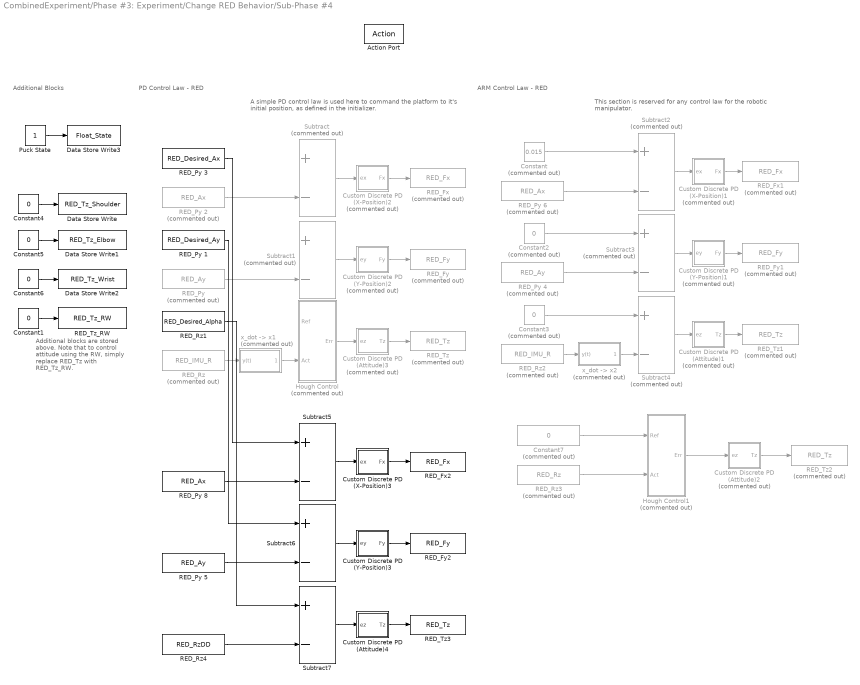
== system CombinedExperiment/Phase #3: Experiment/Change RED Behavior/Sub-Phase #4 ==
  note: ARM Control Law - RED
  note: PD Control Law - RED
  note: Additional Blocks
  note: Additional blocks are stored above. Note that to control attitude using the RW, simply replace RED_Tz with RED_Tz_RW.
  note: A simple PD control law is used here to command the platform to it's initial position, as defined in the initializer.
  note: This section is reserved for any control law for the robotic manipulator.
  Action Port : ActionPort  ActionPortLabel=elseif( u1 < u5)
  Constant : Constant  Commented=on  Value=0.015
  Constant{1,4..6} (4 alike) : Constant  Value=0
  Constant2 : Constant  Commented=on  Value=0
  Constant3 : Constant  Commented=on  Value=0
  Constant7 : Constant  Commented=on  Value=0
  Custom Discrete PD (Attitude)1 : Subsystem  Commented=on
  Custom Discrete PD (Attitude)2 : Subsystem  Commented=on
  Custom Discrete PD (Attitude)3 : Subsystem  Commented=on
  Custom Discrete PD (Attitude)4 : Subsystem
  Custom Discrete PD (X-Position)1 : Subsystem  Commented=on
  Custom Discrete PD (X-Position)2 : Subsystem  Commented=on
  Custom Discrete PD (X-Position)3 : Subsystem
  Custom Discrete PD (Y-Position)1 : Subsystem  Commented=on
  Custom Discrete PD (Y-Position)2 : Subsystem  Commented=on
  Custom Discrete PD (Y-Position)3 : Subsystem
  Data Store Write : DataStoreWrite  DataStoreName=RED_Tz_Shoulder
  Data Store Write1 : DataStoreWrite  DataStoreName=RED_Tz_Elbow
  Data Store Write2 : DataStoreWrite  DataStoreName=RED_Tz_Wrist
  Data Store Write3 : DataStoreWrite  DataStoreName=Float_State
  Hough Control : Subsystem  Commented=on
  Hough Control1 : Subsystem  Commented=on
  Puck State : Constant
  RED_Fx : DataStoreWrite  Commented=on  DataStoreName=RED_Fx
  RED_Fx1 : DataStoreWrite  Commented=on  DataStoreName=RED_Fx
  RED_Fx2 : DataStoreWrite  DataStoreName=RED_Fx
  RED_Fy : DataStoreWrite  Commented=on  DataStoreName=RED_Fy
  RED_Fy1 : DataStoreWrite  Commented=on  DataStoreName=RED_Fy
  RED_Fy2 : DataStoreWrite  DataStoreName=RED_Fy
  "RED_Py " : DataStoreRead  Commented=on  DataStoreName=RED_Ay
  RED_Py 1 : DataStoreRead  DataStoreName=RED_Desired_Ay
  RED_Py 2 : DataStoreRead  Commented=on  DataStoreName=RED_Ax
  RED_Py 3 : DataStoreRead  DataStoreName=RED_Desired_Ax
  RED_Py 4 : DataStoreRead  Commented=on  DataStoreName=RED_Ay
  RED_Py 5 : DataStoreRead  DataStoreName=RED_Ay
  RED_Py 6 : DataStoreRead  Commented=on  DataStoreName=RED_Ax
  RED_Py 8 : DataStoreRead  DataStoreName=RED_Ax
  RED_Rz : DataStoreRead  Commented=on  DataStoreName=RED_IMU_R
  RED_Rz1 : DataStoreRead  DataStoreName=RED_Desired_Alpha
  RED_Rz2 : DataStoreRead  Commented=on  DataStoreName=RED_IMU_R
  RED_Rz3 : DataStoreRead  Commented=on  DataStoreName=RED_Rz
  RED_Rz4 : DataStoreRead  DataStoreName=RED_RzDD
  RED_Tz : DataStoreWrite  Commented=on  DataStoreName=RED_Tz
  RED_Tz1 : DataStoreWrite  Commented=on  DataStoreName=RED_Tz
  RED_Tz2 : DataStoreWrite  Commented=on  DataStoreName=RED_Tz
  RED_Tz3 : DataStoreWrite  DataStoreName=RED_Tz
  RED_Tz_RW : DataStoreWrite  DataStoreName=RED_Tz_RW
  Subtract{,1..4} (5 alike) : Sum  Commented=on  Inputs=+-
  Subtract5 : Sum  Inputs=+-
  Subtract6 : Sum  Inputs=+-
  Subtract7 : Sum  Inputs=+-
  "x_dot -> x1" : Subsystem  Commented=on
  "x_dot -> x2" : Subsystem  Commented=on
  wires:
  Constant1/1 -> RED_Tz_RW/1
  Constant6/1 -> Data Store Write2/1
  Constant4/1 -> Data Store Write/1
  Constant5/1 -> Data Store Write1/1
  RED_Rz/1 -> "x_dot -> x1"/1(y(t))
  Subtract/1 -> Custom Discrete PD (X-Position)2/1(ex)
  Custom Discrete PD (X-Position)2/1(Fx) -> RED_Fx/1
  Custom Discrete PD (Y-Position)2/1(Fy) -> RED_Fy/1
  Custom Discrete PD (Attitude)3/1(Tz) -> RED_Tz/1
  "RED_Py "/1 -> Subtract1/2
  Hough Control/1(Err) -> Custom Discrete PD (Attitude)3/1(ez)
  Subtract1/1 -> Custom Discrete PD (Y-Position)2/1(ey)
  Puck State/1 -> Data Store Write3/1
  "x_dot -> x1"/1(dy(t)/dt) -> Hough Control/2(Act)
  RED_Py 2/1 -> Subtract/2
  Constant2/1 -> Subtract3/1
  "x_dot -> x2"/1(dy(t)/dt) -> Subtract4/2
  Subtract3/1 -> Custom Discrete PD (Y-Position)1/1(ey)
  Constant3/1 -> Subtract4/1
  RED_Py 4/1 -> Subtract3/2
  RED_Rz2/1 -> "x_dot -> x2"/1(y(t))
  Custom Discrete PD (Attitude)1/1(Tz) -> RED_Tz1/1
  RED_Py 6/1 -> Subtract2/2
  Subtract2/1 -> Custom Discrete PD (X-Position)1/1(ex)
  Custom Discrete PD (X-Position)1/1(Fx) -> RED_Fx1/1
  Subtract4/1 -> Custom Discrete PD (Attitude)1/1(ez)
  Constant/1 -> Subtract2/1
  Custom Discrete PD (Y-Position)1/1(Fy) -> RED_Fy1/1
  Hough Control1/1(Err) -> Custom Discrete PD (Attitude)2/1(ez)
  Constant7/1 -> Hough Control1/1(Ref)
  RED_Rz3/1 -> Hough Control1/2(Act)
  Custom Discrete PD (Attitude)2/1(Tz) -> RED_Tz2/1
  Custom Discrete PD (Attitude)4/1(Tz) -> RED_Tz3/1
  Custom Discrete PD (Y-Position)3/1(Fy) -> RED_Fy2/1
  Custom Discrete PD (X-Position)3/1(Fx) -> RED_Fx2/1
  Subtract6/1 -> Custom Discrete PD (Y-Position)3/1(ey)
  Subtract5/1 -> Custom Discrete PD (X-Position)3/1(ex)
  RED_Py 8/1 -> Subtract5/2
  RED_Rz4/1 -> Subtract7/2
  Subtract7/1 -> Custom Discrete PD (Attitude)4/1(ez)
  RED_Py 5/1 -> Subtract6/2
  RED_Py 3/1 -> Subtract5/1
  RED_Py 1/1 -> Subtract6/1
  RED_Rz1/1 -> Subtract7/1

== system CombinedExperiment/Phase #3: Experiment/Change RED Behavior/Subsystem ==
  Universal_Time : DataStoreRead  DataStoreName=Univ_Time
  Time : Outport  VectorParamsAs1DForOutWhenUnconnected=off
  wires:
  Universal_Time/1 -> Time/1

== system CombinedExperiment/Phase #4: Return Home/Change BLACK Behavior/Custom Discrete PD (Attitude) ==
  ez : Inport
  Sum3 : Sum
  kd_tb : Gain  Gain=Kd_tb
  kp_tb : Gain  Gain=Kp_tb
  "x_dot -> x1" : Subsystem
  Tz : Outport  VectorParamsAs1DForOutWhenUnconnected=off
  wires:
  kd_tb/1 -> Sum3/1
  Sum3/1 -> Tz/1
  kp_tb/1 -> Sum3/2
  "x_dot -> x1"/1(dy(t)/dt) -> kd_tb/1
  ez/1 -> "x_dot -> x1"/1(y(t)), kp_tb/1

== system CombinedExperiment/Phase #4: Return Home/Change BLACK Behavior/Custom Discrete PD (X-Position) ==
  ex : Inport
  Sum3 : Sum
  kd_xb : Gain  Gain=Kd_xb
  kp_xb : Gain  Gain=Kp_xb
  "x_dot -> x1" : Subsystem
  Fx : Outport  VectorParamsAs1DForOutWhenUnconnected=off
  wires:
  kd_xb/1 -> Sum3/1
  ex/1 -> "x_dot -> x1"/1(y(t)), kp_xb/1
  kp_xb/1 -> Sum3/2
  "x_dot -> x1"/1(dy(t)/dt) -> kd_xb/1
  Sum3/1 -> Fx/1

== system CombinedExperiment/Phase #4: Return Home/Change BLACK Behavior/Custom Discrete PD (Y-Position) ==
  ey : Inport
  Sum3 : Sum
  kd_yb : Gain  Gain=Kd_yb
  kp_yb : Gain  Gain=Kp_yb
  "x_dot -> x1" : Subsystem
  Fy : Outport  VectorParamsAs1DForOutWhenUnconnected=off
  wires:
  kd_yb/1 -> Sum3/1
  Sum3/1 -> Fy/1
  kp_yb/1 -> Sum3/2
  "x_dot -> x1"/1(dy(t)/dt) -> kd_yb/1
  ey/1 -> "x_dot -> x1"/1(y(t)), kp_yb/1

== system CombinedExperiment/Phase #4: Return Home/Change BLACK Behavior/Hough Control ==
  Ref : Inport
  Act : Inport  Port=2
  MATLAB Function2 : MATLAB Function  TreatAsAtomicUnit=on
  MATLAB Function3 : MATLAB Function  TreatAsAtomicUnit=on
  MATLAB Function4 : MATLAB Function  TreatAsAtomicUnit=on
  Subtract2 : Sum  Inputs=+-
  Err : Outport  VectorParamsAs1DForOutWhenUnconnected=off
  wires:
  MATLAB Function4/1(e_out) -> Err/1
  MATLAB Function2/1(Oy) -> MATLAB Function4/1(Oy)
  Subtract2/1 -> MATLAB Function4/2(e_in)
  MATLAB Function2/2(Ox) -> Subtract2/1
  Act/1 -> MATLAB Function3/1(z)
  Ref/1 -> MATLAB Function2/1(z)
  MATLAB Function3/1(Ox) -> Subtract2/2
